simulink model "HIL_XPlaneMCU"  (R2026b)
settings: Solver=ode4  StopTime=82  FixedStep=0.005  MaxStep=0.05  MinStep=1e-8  AbsTol=1e-4
StartFcn:
  | ins_initial_state_xplane;
undefined symbols (not defined in the file or in its folder): sensors, Ts_xplane
(part 2 of 2)

== matlab function HIL_XPlaneMCU/X-Plane Sensors ==
  settings: updateMethod=DISCRETE  sampleTime=0.05
  data: xplane_sensors output; t input
function xplane_sensors = read_xplane_block(t)

% 1. Todas as declaracoes coder.extrinsic DEVEM ficar aqui no topo
coder.extrinsic('ins_read_xplane');
coder.extrinsic('evalin');

persistent y_last k_last Ts_xplane

% 2. Inicializacao das variaveis persistentes com pre-alocacao de tipo
if isempty(y_last)
    y_last = zeros(1, 18);
end

if isempty(Ts_xplane)
    Ts_xplane = 0.05; % Pre-alocacao default para o Coder saber o tipo (double)
    Ts_xplane = evalin('base', 'Ts_xplane');
end

if isempty(k_last)
    k_last = -1;
end

% Indice discreto da interface X-Plane
k_now = floor(t / Ts_xplane + 1e-9);

% Por padrao, mantem a ultima leitura
xplane_sensors = y_last;

% So le do X-Plane uma vez a cada Ts_xplane
if k_now > k_last
    tmp = zeros(1, 18);
    tmp = ins_read_xplane(0);

    y_last = tmp;
    xplane_sensors = y_last;

    k_last = k_now;
end
end

== matlab function HIL_XPlaneMCU/Navigation/Error_Modeling/ICM20689/gyro_core ==
  data: omega_meas_dps output double size=[3 1]; omega_true_dps input; T input; noise_dps input
function omega_meas_dps = gyro_core(omega_true_dps, T, noise_dps)
%#codegen

coder.extrinsic('ins_gyro_errors_icm20689');
coder.extrinsic('evalin');
sensors = evalin('base', 'sensors');
omega_meas_dps = zeros(3,1);
tmp = zeros(3,1);
tmp = ins_gyro_errors_icm20689(omega_true_dps, T, noise_dps, sensors);

omega_meas_dps = tmp;
end

== matlab function HIL_XPlaneMCU/hil_io ==
  data: t input
function hil_io(t)
%#codegen
coder.extrinsic('hil_serial_udp');
hil_serial_udp(t);

== matlab function HIL_XPlaneMCU/Navigation/Error_Modeling/ICM20689/acc_core ==
  data: acc_true_ms2 input double size=[3 1]; T input double size=[1 1]; noise_ms2 input; acc_meas_ms2 output double size=[3 1]
function acc_meas_ms2 = acc_core(acc_true_ms2, T, noise_ms2)
%#codegen

coder.extrinsic('ins_acc_errors_icm20689');
coder.extrinsic('evalin');

sensors = evalin('base', 'sensors');

acc_meas_ms2 = zeros(3,1);
tmp = zeros(3,1);

tmp = ins_acc_errors_icm20689(acc_true_ms2, T, noise_ms2, sensors);

acc_meas_ms2 = tmp;

end

== matlab function HIL_XPlaneMCU/Navigation/DBN/MATLAB Function ==
  data: acc_b_in input; euler_out output; gyro_b_in input; reset input; sample_valid input; t_now input; vel_out output; pos_out output; acc_n_out output; qb_out output
function [euler_out, vel_out, pos_out, acc_n_out, qb_out] = DBN_block( ...
    acc_b_in, gyro_b_in, reset, sample_valid, t_now)
%#codegen

coder.extrinsic('DBN_solver');
coder.extrinsic('evalin');

euler_out = zeros(3,1);
vel_out   = zeros(3,1);
pos_out   = zeros(3,1);
acc_n_out = zeros(3,1);
qb_out    = zeros(4,1);

DBN_params = evalin('base', 'DBN_params');

euler_tmp = zeros(3,1);
vel_tmp   = zeros(3,1);
pos_tmp   = zeros(3,1);
acc_tmp   = zeros(3,1);
qb_tmp    = zeros(4,1);

[euler_tmp, vel_tmp, pos_tmp, acc_tmp, qb_tmp] = DBN_solver( ...
    acc_b_in, gyro_b_in, reset, sample_valid, t_now, DBN_params);

euler_out = euler_tmp;
vel_out   = vel_tmp;
pos_out   = pos_tmp;
acc_n_out = acc_tmp;
qb_out    = qb_tmp;

end

== matlab function HIL_XPlaneMCU/Navigation/DBN/MATLAB Function1 ==
  data: acc_b_in input; euler_out output; gyro_b_in input; reset input; sample_valid input; t_now input; vel_out output; pos_out output; acc_n_out output; qb_out output
function [euler_out, vel_out, pos_out, acc_n_out, qb_out] = DBN_block_with_error_model( ...
    acc_b_in, gyro_b_in, reset, sample_valid, t_now)
%#codegen

coder.extrinsic('DBN_solver');
coder.extrinsic('evalin');

euler_out = zeros(3,1);
vel_out   = zeros(3,1);
pos_out   = zeros(3,1);
acc_n_out = zeros(3,1);
qb_out    = zeros(4,1);

DBN_params = evalin('base', 'DBN_params');

euler_tmp = zeros(3,1);
vel_tmp   = zeros(3,1);
pos_tmp   = zeros(3,1);
acc_tmp   = zeros(3,1);
qb_tmp    = zeros(4,1);

[euler_tmp, vel_tmp, pos_tmp, acc_tmp, qb_tmp] = DBN_solver( ...
    acc_b_in, gyro_b_in, reset, sample_valid, t_now, DBN_params);

euler_out = euler_tmp;
vel_out   = vel_tmp;
pos_out   = pos_tmp;
acc_n_out = acc_tmp;
qb_out    = qb_tmp;

end

== matlab function HIL_XPlaneMCU/Navigation/EKFs/EKF_DIRETO ==
  data: acc_b_in input; euler_out output; vel_out output; pos_out output; gyro_b_in input; pos_meas_in input; vel_meas_in input; eul_meas_in input; reset input; sample_valid input; t_now input; acc_n_out output; xhat_out output
function [euler_out, vel_out, pos_out, acc_n_out, xhat_out] = EKF_DI_block( ...
    acc_b_in, gyro_b_in, pos_meas_in, vel_meas_in, eul_meas_in, reset, sample_valid, t_now)
%#codegen

coder.extrinsic('EKF_DI_solver');
coder.extrinsic('evalin');

%% Saídas com dimensão fixa

euler_out = zeros(3,1);
vel_out   = zeros(3,1);
pos_out   = zeros(3,1);
acc_n_out = zeros(3,1);
xhat_out  = zeros(21,1);

%% Variáveis temporárias com dimensão fixa

euler_tmp = zeros(3,1);
vel_tmp   = zeros(3,1);
pos_tmp   = zeros(3,1);
acc_tmp   = zeros(3,1);
xhat_tmp  = zeros(21,1);

%% Carrega parâmetros do workspace

EKF_DI_params = evalin('base', 'EKF_DI_params');

%% Chama solver externo

[euler_tmp, vel_tmp, pos_tmp, acc_tmp, xhat_tmp] = EKF_DI_solver( ...
    acc_b_in, gyro_b_in, pos_meas_in, vel_meas_in, eul_meas_in, ...
    reset, sample_valid, t_now, EKF_DI_params);

%% Cópia elemento a elemento para forçar dimensão no Simulink

euler_out(1) = euler_tmp(1);
euler_out(2) = euler_tmp(2);
euler_out(3) = euler_tmp(3);

vel_out(1) = vel_tmp(1);
vel_out(2) = vel_tmp(2);
vel_out(3) = vel_tmp(3);

pos_out(1) = pos_tmp(1);
pos_out(2) = pos_tmp(2);
pos_out(3) = pos_tmp(3);

acc_n_out(1) = acc_tmp(1);
acc_n_out(2) = acc_tmp(2);
acc_n_out(3) = acc_tmp(3);

for k = 1:21
    xhat_out(k) = xhat_tmp(k);
end

end

== matlab function HIL_XPlaneMCU/Navigation/EKFs/MATLAB Function ==
  data: vN input; VT output; vE input; vD input
function VT  = true_air_speed(vN, vE, vD)
    VT = sqrt(vN^2 + vE^2 + vD^2);
end
